simulink model "huizhenglijujisuan_zuixin"  (R2024b)
settings: Solver=FixedStepAuto  StartTime=0.0  StopTime=10  FixedStep=1e-4  MaxStep=1e-2  RelTol=1e-3
model workspace (MAT data in the model file):
  angle = Simulink.Parameter
  angle.Value = [-0.500377774 -0.503118992 -0.475854188 -0.406988144 -0.304092586 -0.178856105 -0.040153947 0.103196472 0.244897678 0.381538063 0.512861133 0.642340958 ... (2682 elements, 2682x1)]
  angle.Complexity = 'real'
  angle.Dimensions = [2682 1]
  angle.DataType = 'auto'
libraries: simulink x4, spsPermanentMagnetSynchronousMachineLib x2, slpidlib x2, powerlib_extras x2, Solver_SF x1, spsDCVoltageSourceLib x1, spsUniversalBridgeLib x1, spspowerguiLib x1
(part 1 of 2)
settings Model: Creator=L大锤  LastModifiedBy=L大锤
settings DataIOCC: ExternalInput=[t, a]
settings ModelReferenceCC: EnableRefExpFcnMdlSchedulingChecks=on
settings RTWCC: GPUComputeCapability=3.5

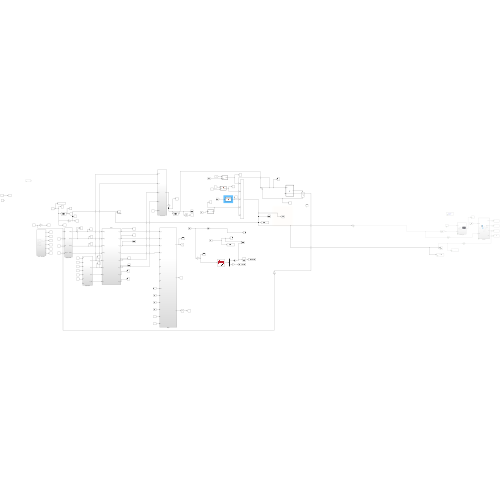
[thumbnail: Simulink's stored preview of the top-level diagram]
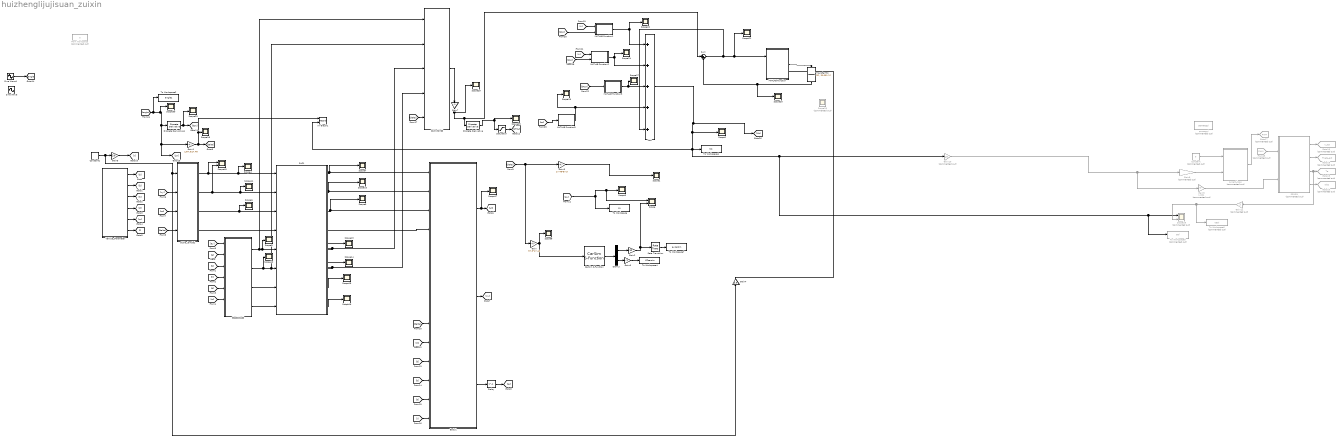
== system huizhenglijujisuan_zuixin ==
  Add : Sum  Inputs=+++++
  Body1 : Subsystem
  CarSim S-Function : Solver_SF/CarSim S-Function  Priority=1  SIMFILE=simfile.sim  Run_RTs=off  vs_state_ind=Run  StopMode_ind=Vehicle Model
  Constant : Constant  Commented=on  Value=0
  Constant1 : Constant  Value=80/3.6
  Delay : Delay  DelayLength=1
  Demux : Demux  Outputs=2
  Discrete Derivative : simulink/Quick Insert/Discrete/Discrete Derivative  gainval=1.0  ICPrevScaledInput=0.0  OutMin=[]  OutMax=[10]  OutDataType=fixdt(1, 16)  OutScaling=2^-10  DoSatur=on
  Discrete Derivative1 : simulink/Quick Insert/Discrete/Discrete Derivative  gainval=1.0  ICPrevScaledInput=0.0  OutMin=[]  OutMax=[]  OutDataType=fixdt(1, 16)  OutScaling=2^-10  DoSatur=off
  From Workspace : FromWorkspace  Commented=on  VariableName=a  OutDataTypeStr=double  SampleTime=0.001  Interpolate=off  OutputAfterFinalValue=Setting to zero
  From25 : From  Commented=on  GotoTag=PWM  TagVisibility=global
  Gain : Gain  Gain=57.3*17.48
  Gain1 : Gain  Gain=1/57.3/17.48
  Gain10 : Gain  Commented=on  Gain=1/3
  Gain11 : Gain  Commented=on  Gain=3
  Gain2 : Gain  Gain=10
  Gain3 : Gain  Gain=17.48*57.3
  Gain4 : Gain  Gain=3.6
  Gain5 : Gain  Gain=3.6
  Gain6 : Gain  Gain=-1
  Gain7 : Gain  Gain=-1
  Gain8 : Gain  Commented=on  Gain=1/0.11247
  Gain9 : Gain  Commented=on  Gain=1.001
  Goto15 : Goto  Commented=on  GotoTag=n_act  TagVisibility=global
  Goto16 : Goto  Commented=on  GotoTag=Iabc  TagVisibility=global
  Goto17 : Goto  Commented=on  GotoTag=PWM  TagVisibility=global
  Goto18 : Goto  Commented=on  GotoTag=Theta_act  TagVisibility=global
  Goto19 : Goto  Commented=on  GotoTag=Te  TagVisibility=global
  MATLAB Function : MATLAB Function  TreatAsAtomicUnit=on
  MATLAB Function1 : MATLAB Function  TreatAsAtomicUnit=on
  MATLAB Function2 : MATLAB Function  TreatAsAtomicUnit=on
  MATLAB Function3 : MATLAB Function  TreatAsAtomicUnit=on
  MATLAB Function5 : MATLAB Function  TreatAsAtomicUnit=on
  PAC1 : Subsystem
  Rate Transition : RateTransition
  SPMSM : Subsystem  Commented=on
  Saturation : Saturate  UpperLimit=10  LowerLimit=-10
  Scope : Scope  NumInputPorts=2
  Scope{1..25,27,29..30} (28 alike) : Scope
  Scope26 : Scope  Commented=on
  Scope28 : Scope  Commented=on  NumInputPorts=2
  Scope48 : Scope  NumInputPorts=2
  Sine Wave : Sin  Amplitude=400  Frequency=2*pi/10  SampleTime=0
  Sine Wave1 : Sin  Amplitude=20  Frequency=2*pi/5  SampleTime=0
  Sum : Sum  Inputs=|+-
  To Workspace : ToWorkspace  VariableName=ay  SampleTime=-1
  To Workspace1 : ToWorkspace  VariableName=MZ  SampleTime=-1
  To Workspace2 : ToWorkspace  VariableName=angle1  SampleTime=-1
  To Workspace4 : ToWorkspace  VariableName=MZcarsim  SampleTime=-1
  To Workspace5 : ToWorkspace  Commented=on  VariableName=tref  SampleTime=-1
  To Workspace6 : ToWorkspace  Commented=on  VariableName=treal  SampleTime=-1
  To Workspace7 : ToWorkspace  VariableName=aycarsim  SampleTime=-1
  Transfer Fcn : TransferFcn  Denominator=[0.001 1]
  Vehicle_Parameter : Subsystem
  XY Graph1 : Record  FileSettingsInternal="{\"entries\":[{\"content\":{\"excelSettings\":{\"content\":{},\"type\":\"Streamout.ExcelSettings\"}},\"type\":\"Streamout.FileSettingStorage\",\"uuid\":\"\"}],\"packageUris\":[\"http:\\/\\/schema.mathworks.com\\/mf0\\/streamout_blocks\\/R2020a\"],\"version\":\"1.0\"}"  Layout=[1 1]  SignalsInternal="{\"entries\":[{\"content\":{\"signals\":[{\"content\":{\"blockPath\":[],\"dimensions\":[1],\"domain\":\"\",\"lineColor\":\"#edb120\",\"lineWidth\":2,\"port\":1,\"sid\":[\"\"],\"signalID\":1,\"signalName\":\"Gain1\"},\"type\":\"RecordBlkView.Signal\",\"uuid\":\"\"},{\"content\":{\"blockPath\":[],\"dimensions\":[1],\"domain\":\"\",\"lineColor\":\"#7e2f8e\",\"lineWidth\":2,\"port\":2,\"sid\":[\"\"],\"signalID\":2,\"signalName\":\"Add\"},\"type\":\"RecordBlkView.Signal\",\"uuid\":\"\"}]},\"type\":\"RecordBlkView.InputSignals\",\"uuid\":\"\"}],\"packageUris\":[\"http:\\/\\/schema.mathworks.com\\/mf0\\/streamout_blocks\\/R2020a\"],\"version\":\"1.0\"}"  VisualizationBindings="{\"xyplotplugin\":{\"info\":[{\"series\":[],\"subplotID\":1}]}}"  CompatibilityTag=XY
  alpha_lamda1 : Subsystem
  current_loop : Subsystem  Commented=on
  powergui : spspowerguiLib/powergui  Priority=1  Commented=on  SimulationMode=Discrete  SampleTime=1/2000/500  frequency=60  Iterations=50  frequencyindice=0  Pbase=100e6  ErrMax=1e-4  UnitsV=kV  UnitsW=MW  buscounter=0  FunctionMessages=off  echomessages=off  EnableUseOfTLC=off  CurrentSourceSwitches=off  DisableSnubberDevices=off  DisableRonSwitches=off  DisableVfSwitches=off  DisplayEquations=off  AutomaticDiscreteSolvers=off  SolverType=Tustin/Backward Euler (TBE)  Interpol=off  ExternalGateDelay=off  methode=off  Ts=100  x0status=blocks  SPID=on  SwTol=0  HookPort=off  NonlinearTolerance=1e-4  nMaxIteration=100  ContinueOnMaxIteration=off  RestoreLinks=warning  ResistiveCurrentMeasurement=off  Frange=[0:2:500]  Ylog=off  Xlog=on  ShowGrid=off  save=off  variable=ZData  structure=ia  ZoomFFT=off  StartTime=.775  cycles=1  DisplayStyle=1  fundamental=400  FreqAxis=off  MaxFrequency=40000  frequencyindicesteady=1  RmsSteady=1  display=off
  回正力矩计算 : Subsystem
  垂直载荷估算 : Subsystem
  wires:
  alpha_lamda1/1(alpha_fl) -> Scope48/1, Scope4/1, PAC1/1(alpha_fl)
  alpha_lamda1/2(alpha_fr) -> Scope48/2, Scope11/1, PAC1/2(alpha_fr)
  alpha_lamda1/4(alpha_rr) -> PAC1/4(alpha_rr)
  垂直载荷估算/3(Fz_L2) -> PAC1/7(Fz_rl)
  垂直载荷估算/4(Fz_R2) -> PAC1/8(Fz_rr)
  垂直载荷估算/2(Fz_fr) -> 回正力矩计算/2(Fz_fr), PAC1/6(Fz_fr), Scope12/1
  垂直载荷估算/1(Fz_fl) -> 回正力矩计算/1(Fz_fl), PAC1/5(Fz_fl), Scope5/1
  PAC1/1(Fy_fl) -> Scope7/1, Body1/1(Fy_fl)
  PAC1/2(Fy_fr) -> Scope10/1, Body1/2(Fy_fr)
  PAC1/3(Fy_rl) -> Scope9/1, Body1/3(Fy_rl)
  PAC1/4(Fy_rr) -> Body1/4(Fy_rr)
  Gain/1 -> CarSim S-Function/1, Scope8/1
  PAC1/5(Mz_fl) -> Scope13/1, 回正力矩计算/3(M_fl)
  PAC1/6(Mz_fr) -> Scope14/1, 回正力矩计算/4(M_fr)
  Gain3/1 -> Scope1/1
  Body1/3(ay) -> Delay/1
  alpha_lamda1/3(alpha_rl) -> Scope6/1, PAC1/3(alpha_rl)
  PAC1/7(Mz_rl) -> Scope15/1
  PAC1/8(Mz_rr) -> Scope16/1
  Vehicle_Parameter/1(a) -> [a]
  Vehicle_Parameter/2(b) -> [b]
  Vehicle_Parameter/3(h) -> [h]
  Vehicle_Parameter/4(d) -> [d]
  Vehicle_Parameter/5(m) -> [m]
  Vehicle_Parameter/6(l) -> [I]
  [a] -> 垂直载荷估算/2(a)
  [b] -> 垂直载荷估算/3(b)
  [h] -> 垂直载荷估算/4(h)
  [d] -> 垂直载荷估算/5(d)
  [m] -> 垂直载荷估算/6(m)
  [ay] -> 垂直载荷估算/1(Ay)
  [vy] -> alpha_lamda1/2(vy)
  [wz] -> alpha_lamda1/3(wz)
  [delta] -> alpha_lamda1/4(delta_fl)
  Delay/1 -> [ay]
  Body1/2(vy) -> [vy]
  Body1/1(wz) -> Scope17/1, [wz]
  [delta] -> Gain3/1, Gain/1
  [delta] -> Body1/9(delta)
  [ay] -> Scope/1, Scope3/1, To Workspace/1
  [m] -> Body1/10(m)
  [d] -> Body1/11(d)
  [b] -> Body1/12(b)
  [a] -> Body1/13(a)
  [I] -> Body1/14(Iz)
  [delta] -> 回正力矩计算/5(delta)
  Gain1/1 -> XY Graph1/1, Scope18/1, [delta]
  Constant1/1 -> Gain4/1, alpha_lamda1/1(vx), Gain5/1
  Gain4/1 -> MATLAB Function/2(v)
  MATLAB Function/1(Tz) -> Transfer Fcn/1
  Transfer Fcn/1 -> Scope20/1, Sum/2
  Gain5/1 -> [v]
  Discrete Derivative1/1 -> [dsw], Scope23/1
  回正力矩计算/1(Mz) -> Gain7/1
  [sw] -> MATLAB Function5/1(sw)
  Demux/1 -> Gain2/1
  Demux/2 -> Gain6/1
  Gain7/1 -> Scope29/1, Discrete Derivative/1, Sum/1
  Gain6/1 -> To Workspace4/1
  [angle] -> To Workspace2/1, Scope30/1, Discrete Derivative1/1, [sw], Gain1/1
  MATLAB Function5/1(Tlim) -> Scope19/1, Add/4
  CarSim S-Function/1 -> Demux/1
  MATLAB Function3/1(Tguanxing) -> Scope27/1, Add/3
  [v] -> MATLAB Function2/1(v)
  [dsw] -> MATLAB Function2/2(dsw)
  [v] -> MATLAB Function1/1(v)
  MATLAB Function2/1(Tzuni) -> Scope24/1, Add/2
  [dsw] -> MATLAB Function1/2(dsw)
  MATLAB Function1/1(Tfric) -> Add/1, Scope22/1
  [dTsw] -> MATLAB Function3/1(dtsw)
  Sum/1 -> Scope21/1, MATLAB Function/1(Tsw), Add/5
  Discrete Derivative/1 -> Saturation/1, Scope25/1
  Saturation/1 -> [dTsw]
  From25/1 -> SPMSM/1(pwm)
  SPMSM/2(theta_act) -> Goto18/1
  current_loop/1(pwm) -> Goto17/1
  Gain9/1 -> SPMSM/2(load)
  Gain8/1 -> current_loop/2(iq*)
  SPMSM/4(Iabc) -> Goto16/1
  SPMSM/1(n_act) -> Goto15/1
  Constant/1 -> current_loop/1(id*)
  Add/1 -> [Mz], To Workspace5/1, Scope28/1, Gain10/1, XY Graph1/2, To Workspace1/1, Scope2/1
  SPMSM/3(Te) -> Gain11/1, Goto19/1
  Gain10/1 -> Gain9/1, Gain8/1
  Gain11/1 -> To Workspace6/1, Scope28/2
  Gain2/1 -> Rate Transition/1, Scope/2
  Sine Wave1/1 -> [angle]
  Rate Transition/1 -> To Workspace7/1

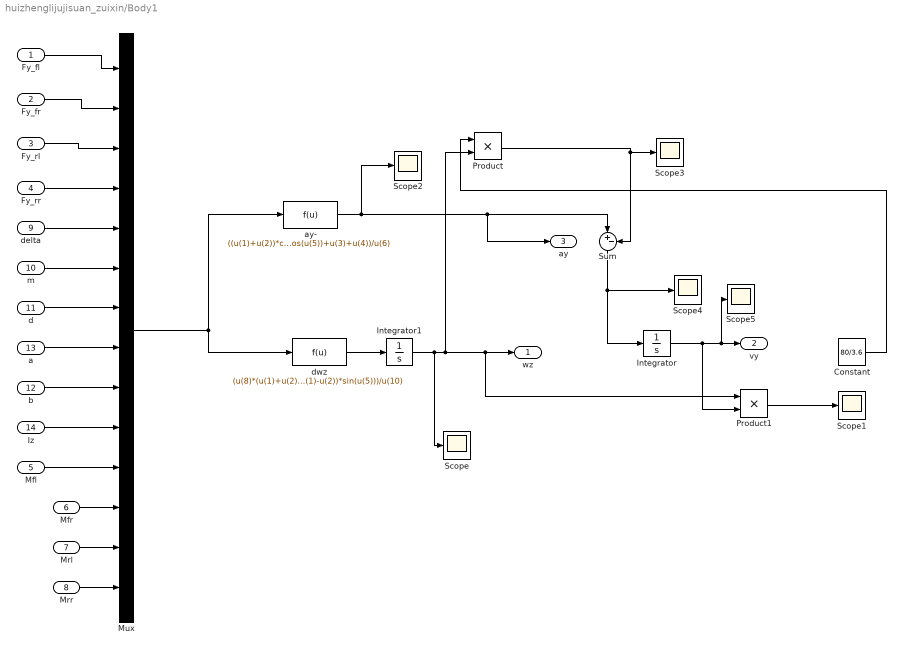
== system huizhenglijujisuan_zuixin/Body1 ==
  Fy_fl : Inport
  Fy_fr : Inport  Port=2
  Fy_rl : Inport  Port=3
  Fy_rr : Inport  Port=4
  Mfl : Inport  Port=5
  Mfr : Inport  Port=6
  Mrl : Inport  Port=7
  Mrr : Inport  Port=8
  delta : Inport  Port=9
  m : Inport  Port=10
  d : Inport  Port=11
  b : Inport  Port=12
  a : Inport  Port=13
  Iz : Inport  Port=14
  Constant : Constant  Value=80/3.6
  Integrator : Integrator
  Integrator1 : Integrator
  Mux : Mux  Inputs=14
  Product : Product
  Product1 : Product
  Scope{,1..5} (6 alike) : Scope
  Sum : Sum  Inputs=|+-
  ay- : Fcn  Expr=((u(1)+u(2))*cos(u(5))+u(3)+u(4))/u(6)
  dwz : Fcn  Expr=(u(8)*(u(1)+u(2))*cos(u(5))-u(9)*(u(3)+u(4))+u(7)/2*(u(1)-u(2))*sin(u(5)))/u(10)
  wz : Outport
  vy : Outport  Port=2
  ay : Outport  Port=3
  wires:
  Mux/1 -> ay-/1, dwz/1
  ay-/1 -> Scope2/1, ay/1, Sum/1
  dwz/1 -> Integrator1/1
  Integrator1/1 -> Scope/1, Product/2, Product1/1, wz/1
  Fy_fl/1 -> Mux/1
  Fy_fr/1 -> Mux/2
  Fy_rl/1 -> Mux/3
  Fy_rr/1 -> Mux/4
  delta/1 -> Mux/5
  m/1 -> Mux/6
  Constant/1 -> Product/1
  Product/1 -> Scope3/1, Sum/2
  Sum/1 -> Scope4/1, Integrator/1
  Integrator/1 -> Product1/2, Scope5/1, vy/1
  Product1/1 -> Scope1/1
  d/1 -> Mux/7
  a/1 -> Mux/8
  b/1 -> Mux/9
  Iz/1 -> Mux/10
  Mfl/1 -> Mux/11
  Mfr/1 -> Mux/12
  Mrl/1 -> Mux/13
  Mrr/1 -> Mux/14

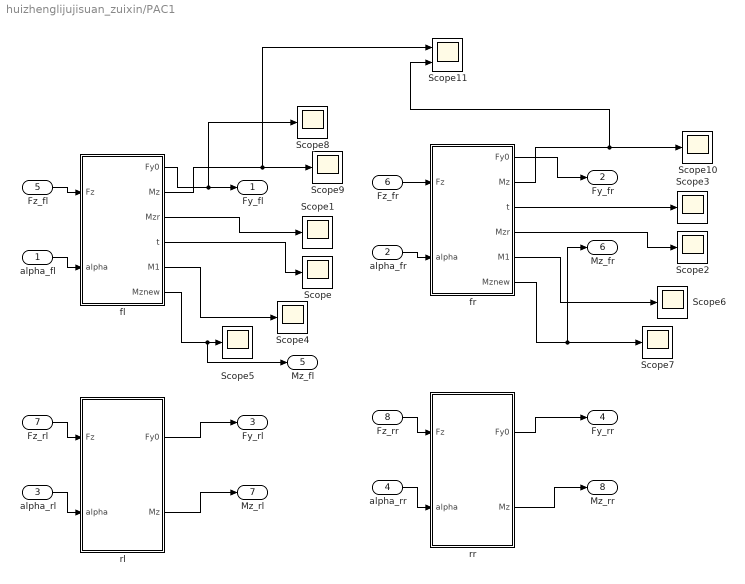
== system huizhenglijujisuan_zuixin/PAC1 ==
  alpha_fl : Inport
  alpha_fr : Inport  Port=2
  alpha_rl : Inport  Port=3
  alpha_rr : Inport  Port=4
  Fz_fl : Inport  Port=5
  Fz_fr : Inport  Port=6
  Fz_rl : Inport  Port=7
  Fz_rr : Inport  Port=8
  Scope{,1..10} (11 alike) : Scope
  Scope11 : Scope  NumInputPorts=2
  fl : MATLAB Function  TreatAsAtomicUnit=on
  fr : MATLAB Function  TreatAsAtomicUnit=on
  rl : MATLAB Function  TreatAsAtomicUnit=on
  rr : MATLAB Function  TreatAsAtomicUnit=on
  Fy_fl : Outport
  Fy_fr : Outport  Port=2
  Fy_rl : Outport  Port=3
  Fy_rr : Outport  Port=4
  Mz_fl : Outport  Port=5
  Mz_fr : Outport  Port=6
  Mz_rl : Outport  Port=7
  Mz_rr : Outport  Port=8
  wires:
  fl/2(Mz) -> Scope11/1, Scope9/1
  Fz_fl/1 -> fl/1(Fz)
  alpha_fl/1 -> fl/2(alpha)
  fl/1(Fy0) -> Scope8/1, Fy_fl/1
  Fz_fr/1 -> fr/1(Fz)
  alpha_fr/1 -> fr/2(alpha)
  fr/1(Fy0) -> Fy_fr/1
  Fz_rl/1 -> rl/1(Fz)
  alpha_rl/1 -> rl/2(alpha)
  rl/1(Fy0) -> Fy_rl/1
  Fz_rr/1 -> rr/1(Fz)
  alpha_rr/1 -> rr/2(alpha)
  rr/2(Mz) -> Mz_rr/1
  rr/1(Fy0) -> Fy_rr/1
  fl/4(t) -> Scope/1
  fl/3(Mzr) -> Scope1/1
  fr/4(Mzr) -> Scope2/1
  fr/3(t) -> Scope3/1
  fl/5(M1) -> Scope4/1
  fl/6(Mznew) -> Mz_fl/1, Scope5/1
  fr/5(M1) -> Scope6/1
  fr/6(Mznew) -> Mz_fr/1, Scope7/1
  fr/2(Mz) -> Scope11/2, Scope10/1
  rl/2(Mz) -> Mz_rl/1

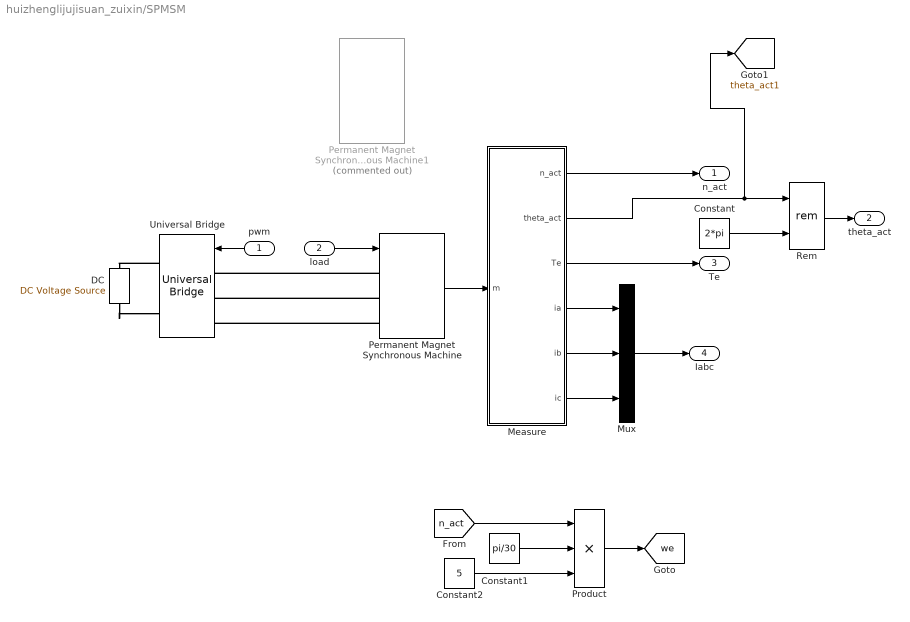
== system huizhenglijujisuan_zuixin/SPMSM ==
  pwm : Inport
  load : Inport  Port=2
  Constant : Constant  Value=2*pi
  Constant1 : Constant  Value=pi/30
  Constant2 : Constant  Value=5
  "DC " : spsDCVoltageSourceLib/DC Voltage Source  Amplitude=200  Measurements=None
  Measure : Subsystem
  Mux : Mux  Inputs=3
  Permanent Magnet Synchronous Machine : spsPermanentMagnetSynchronousMachineLib/Permanent Magnet Synchronous Machine  NbPhases=3  FluxDistribution=Sinusoidal  RotorType=Round  MechanicalLoad=Torque Tm  PresetModel=No  ShowDetailedParameters=on  MeasurementBus=off  Resistance=0.12  Inductance=8.5e-3  dqInductances=[4e-3, 4e-3]  La=0.97e-3  MachineConstant=Voltage Constant (V_peak L-L / krpm)  Flux=0.014996  VoltageCst=13.6  TorqueCst=0.11247  Flat=120  Mechanical=[0.00107 0 5 0]  PolePairs=4  InitialConditions=[0,0, 0,0]  InitialConditions5ph=[0 0 0 0 0 0]  RefAngle=Aligned with phase A axis (original Park)  IterativeDiscreteModel=Trapezoidal non iterative  TsBlock=-1  TsPowergui=0
  Permanent Magnet Synchronous Machine1 : spsPermanentMagnetSynchronousMachineLib/Permanent Magnet Synchronous Machine  Commented=on  NbPhases=3  FluxDistribution=Sinusoidal  RotorType=Salient-pole  MechanicalLoad=Torque Tm  PresetModel=No  ShowDetailedParameters=on  MeasurementBus=off  Resistance=2.875  Inductance=8.5e-3  dqInductances=[4e-3, 4e-3]  La=0.000835  MachineConstant=Flux linkage established by magnets (V.s)  Flux=0.175  VoltageCst=126.966  TorqueCst=1.05  Flat=120  Mechanical=[0.003 0 4 0]  PolePairs=4  InitialConditions=[0,0, 0,0]  InitialConditions5ph=[0 0 0 0 0 0]  RefAngle=Aligned with phase A axis (original Park)  IterativeDiscreteModel=Trapezoidal non iterative  TsBlock=-1  TsPowergui=0
  Product : Product  Inputs=3
  Rem : Math  Operator=rem
  Universal Bridge : spsUniversalBridgeLib/Universal Bridge  Arms=3  SnubberResistance=1e5  SnubberCapacitance=inf  Device=IGBT / Diodes  Ron=1e-3  Lon=0  ForwardVoltages="[  0  0  ]"  ForwardVoltage=0  GTOparameters=[ 10e-6 , 20e-6 ]  IGBTparameters=[ 1e-6 , 2e-6 ]  Measurements=None  Measurements_2=None  converterType=Rectifier
  n_act : Outport
  theta_act : Outport  Port=2
  Te : Outport  Port=3
  Iabc : Outport  Port=4
  tag scope: theta_act1=global, we=global
  wires:
  pwm/1 -> Universal Bridge/1
  load/1 -> Permanent Magnet Synchronous Machine/1
  Permanent Magnet Synchronous Machine/1 -> Measure/1(m)
  Measure/1(n_act) -> n_act/1
  Measure/3(Te) -> Te/1
  Measure/4(ia) -> Mux/1
  Measure/5(ib) -> Mux/2
  Measure/6(ic) -> Mux/3
  Mux/1 -> Iabc/1
  Rem/1 -> theta_act/1
  Constant/1 -> Rem/2
  Measure/2(theta_act) -> [theta_act1], Rem/1
  [n_act] -> Product/1
  Constant1/1 -> Product/2
  Constant2/1 -> Product/3
  Product/1 -> [we]
  connections:
  "DC "/LConn1 -- Universal Bridge/RConn2
  Universal Bridge/RConn1 -- "DC "/RConn1
  Permanent Magnet Synchronous Machine/LConn3 -- Universal Bridge/LConn3
  Permanent Magnet Synchronous Machine/LConn1 -- Universal Bridge/LConn1
  Permanent Magnet Synchronous Machine/LConn2 -- Universal Bridge/LConn2

== system huizhenglijujisuan_zuixin/Vehicle_Parameter ==
  Constant : Constant  Value=2636
  Constant1 : Constant  Value=1.701
  Constant2 : Constant  Value=1.427
  Constant3 : Constant  Value=1.572
  Constant4 : Constant  Value=0.5848
  Constant8 : Constant  Value=4500
  a : Outport
  b : Outport  Port=2
  h : Outport  Port=3
  d : Outport  Port=4
  m : Outport  Port=5
  l : Outport  Port=6
  wires:
  Constant/1 -> m/1
  Constant3/1 -> a/1
  Constant2/1 -> b/1
  Constant4/1 -> h/1
  Constant1/1 -> d/1
  Constant8/1 -> l/1

== system huizhenglijujisuan_zuixin/alpha_lamda1 ==
  vx : Inport
  vy : Inport  Port=2
  wz : Inport  Port=3
  delta_fl : Inport  Port=4
  alpha : Subsystem
  alpha_fl : Outport
  alpha_fr : Outport  Port=2
  alpha_rl : Outport  Port=3
  alpha_rr : Outport  Port=4
  wires:
  alpha/1(alpha_fl) -> alpha_fl/1
  alpha/2(alpha_fr) -> alpha_fr/1
  alpha/3(alpha_rl) -> alpha_rl/1
  alpha/4(alpha_rr) -> alpha_rr/1
  vx/1 -> alpha/1(vx)
  vy/1 -> alpha/2(vy)
  wz/1 -> alpha/3(wz)
  delta_fl/1 -> alpha/4(delta_fl)

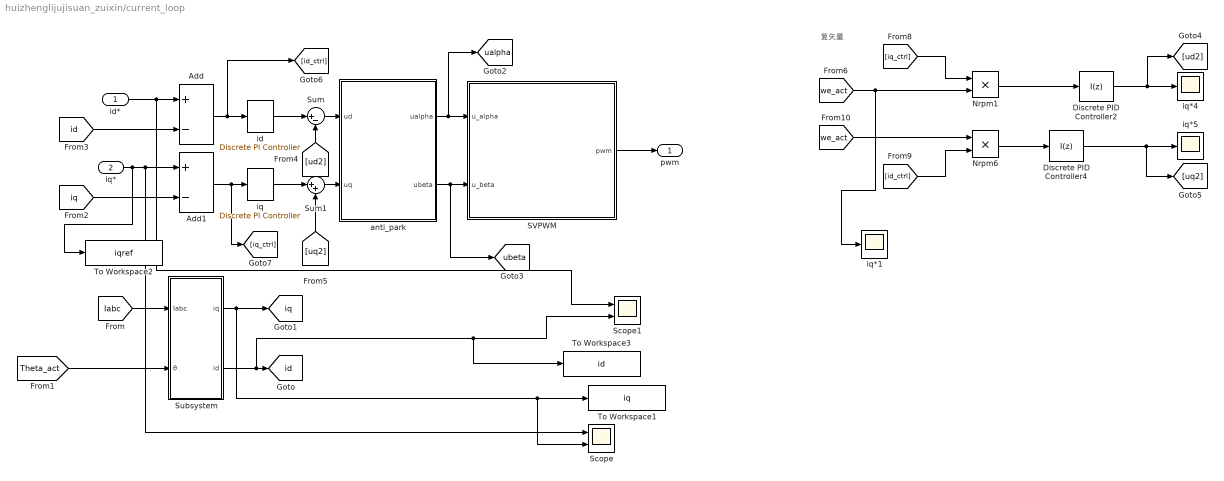
== system huizhenglijujisuan_zuixin/current_loop ==
  note: 复矢量
  id* : Inport
  iq* : Inport  Port=2
  Add : Sum  Inputs=+-
  Add1 : Sum  Inputs=+-
  Discrete PID Controller2 : slpidlib/PID Controller  Controller=I  Form=Parallel  TimeDomain=Discrete-time  UseExternalTs=off  SampleTime=1e-4  IntegratorMethod=Forward Euler  FilterMethod=Forward Euler  ControllerParametersSource=internal  P=0  I=0.32/10000  UseKiTs=off  D=0  UseExternalDerivativeSource=off  N=100  UseFilter=on  TunerSelectOption=Transfer Function Based (PID Tuner App)  InitialConditionSource=internal  InitialConditionForIntegrator=0  InitialConditionForFilter=0  DifferentiatorICPrevScaledInput=0  ExternalReset=none  TrackingMode=off  Kt=1  LimitOutput=on  SatLimitsSource=internal  UpperSaturationLimit=600  LowerSaturationLimit=-600  LinearizeAsGain=off  AntiWindupMode=none  Kb=1  LimitIntegrator=off  UpperIntegratorSaturationLimit=inf  LowerIntegratorSaturationLimit=-inf  POutMin=[]  POutMax=[]  IOutMin=[]  IOutMax=[]  DOutMin=[]  DOutMax=[]  NOutMin=[]  NOutMax=[]  SumOutMin=[]  SumOutMax=[]  SaturationOutMin=[]  SaturationOutMax=[]  PParamMin=[]  PParamMax=[]  IParamMin=[]  IParamMax=[]  DParamMin=[]  DParamMax=[]  NParamMin=[]  NParamMax=[]  KbParamMin=[]  KbParamMax=[]  KtParamMin=[]  KtParamMax=[]  KbOutMin=[]  KbOutMax=[]  KtOutMin=[]  KtOutMax=[]  IntegratorOutMin=[]  IntegratorOutMax=[]  FilterOutMin=[]  FilterOutMax=[]  SumI1OutMin=[]  SumI1OutMax=[]  SumI2OutMin=[]  SumI2OutMax=[]  SumI3OutMin=[]  SumI3OutMax=[]  SumI4OutMin=[]  SumI4OutMax=[]  SumDOutMin=[]  SumDOutMax=[]  DifferentiatorOutMin=[]  DifferentiatorOutMax=[]  FilterDiffOutCoefMin=[]  FilterDiffOutCoefMax=[]  ReciprocalOutMin=[]  ReciprocalOutMax=[]  SumDenOutMin=[]  SumDenOutMax=[]  SumNumOutMin=[]  SumNumOutMax=[]  DivideOutMin=[]  DivideOutMax=[]  UdiffTsProdOutMin=[]  UdiffTsProdOutMax=[]  NTsProdOutMin=[]  NTsProdOutMax=[]  UintegralTsProdOutMin=[]  UintegralTsProdOutMax=[]  UngainTsProdOutMin=[]  UngainTsProdOutMax=[]  ClampingZeroOutDataTypeStr=Inherit: Inherit via back propagation  ClampingZeroOutMin=[]  ClampingZeroOutMax=[]  FilterDenConstantOutDataTypeStr=Inherit: Inherit via back propagation  FilterDenConstantOutMin=[]  FilterDenConstantOutMax=[]  PCopyOutDataTypeStr=Inherit: Inherit via back propagation  PCopyOutMin=[]  PCopyOutMax=[]  NCopyOutDataTypeStr=Inherit: Inherit via back propagation  NCopyOutMin=[]  NCopyOutMax=[]  IntegratorContinuousStateAttributes=''  IntegratorStateMustResolveToSignalObject=off  IntegratorRTWStateStorageClass=Auto  FilterContinuousStateAttributes=''  FilterStateMustResolveToSignalObject=off  FilterRTWStateStorageClass=Auto  ParallelPVariant=Disabled  IdealPVariant=Disabled  IVariant=InternalParameters  DVariant=Disabled  IntegratorVariant=Discrete  SatVariant=Enabled  AWVariant=Passthrough  PCopyVariant=Disabled  TRVariant=Disabled  FdbkBlocksVariant=Forward  IdealPFdbkVariant=Disabled  SatFdbkVariant=Disabled  DerivativeFilterVariant=Disabled  NVariant=Disabled  NCopyVariant=Disabled_SignalSpec  FilterICVariant=Disabled  IntegratorICVariant=InternalICs  ExternalResetVariant=Disabled  TRSumVariant=Passthrough  SumFdbkVariant=Disabled  SumVariant=Passthrough_I  TsampFilterVariant=InternalTs  TsampNgainVariant=Passthrough  TsampIntegralVariant=Disabled_SignalSpec  ExternalSaturationOutDataTypeStr=Inherit: Same as second input  DerivativeSourceVariant=Disabled  PreIntVariant=InternalPreInt
  Discrete PID Controller4 : slpidlib/PID Controller  Controller=I  Form=Parallel  TimeDomain=Discrete-time  UseExternalTs=off  SampleTime=1e-4  IntegratorMethod=Forward Euler  FilterMethod=Forward Euler  ControllerParametersSource=internal  P=0  I=0.32/10000  UseKiTs=off  D=0  UseExternalDerivativeSource=off  N=100  UseFilter=on  TunerSelectOption=Transfer Function Based (PID Tuner App)  InitialConditionSource=internal  InitialConditionForIntegrator=0  InitialConditionForFilter=0  DifferentiatorICPrevScaledInput=0  ExternalReset=none  TrackingMode=off  Kt=1  LimitOutput=on  SatLimitsSource=internal  UpperSaturationLimit=600  LowerSaturationLimit=-600  LinearizeAsGain=off  AntiWindupMode=none  Kb=1  LimitIntegrator=off  UpperIntegratorSaturationLimit=inf  LowerIntegratorSaturationLimit=-inf  POutMin=[]  POutMax=[]  IOutMin=[]  IOutMax=[]  DOutMin=[]  DOutMax=[]  NOutMin=[]  NOutMax=[]  SumOutMin=[]  SumOutMax=[]  SaturationOutMin=[]  SaturationOutMax=[]  PParamMin=[]  PParamMax=[]  IParamMin=[]  IParamMax=[]  DParamMin=[]  DParamMax=[]  NParamMin=[]  NParamMax=[]  KbParamMin=[]  KbParamMax=[]  KtParamMin=[]  KtParamMax=[]  KbOutMin=[]  KbOutMax=[]  KtOutMin=[]  KtOutMax=[]  IntegratorOutMin=[]  IntegratorOutMax=[]  FilterOutMin=[]  FilterOutMax=[]  SumI1OutMin=[]  SumI1OutMax=[]  SumI2OutMin=[]  SumI2OutMax=[]  SumI3OutMin=[]  SumI3OutMax=[]  SumI4OutMin=[]  SumI4OutMax=[]  SumDOutMin=[]  SumDOutMax=[]  DifferentiatorOutMin=[]  DifferentiatorOutMax=[]  FilterDiffOutCoefMin=[]  FilterDiffOutCoefMax=[]  ReciprocalOutMin=[]  ReciprocalOutMax=[]  SumDenOutMin=[]  SumDenOutMax=[]  SumNumOutMin=[]  SumNumOutMax=[]  DivideOutMin=[]  DivideOutMax=[]  UdiffTsProdOutMin=[]  UdiffTsProdOutMax=[]  NTsProdOutMin=[]  NTsProdOutMax=[]  UintegralTsProdOutMin=[]  UintegralTsProdOutMax=[]  UngainTsProdOutMin=[]  UngainTsProdOutMax=[]  ClampingZeroOutDataTypeStr=Inherit: Inherit via back propagation  ClampingZeroOutMin=[]  ClampingZeroOutMax=[]  FilterDenConstantOutDataTypeStr=Inherit: Inherit via back propagation  FilterDenConstantOutMin=[]  FilterDenConstantOutMax=[]  PCopyOutDataTypeStr=Inherit: Inherit via back propagation  PCopyOutMin=[]  PCopyOutMax=[]  NCopyOutDataTypeStr=Inherit: Inherit via back propagation  NCopyOutMin=[]  NCopyOutMax=[]  IntegratorContinuousStateAttributes=''  IntegratorStateMustResolveToSignalObject=off  IntegratorRTWStateStorageClass=Auto  FilterContinuousStateAttributes=''  FilterStateMustResolveToSignalObject=off  FilterRTWStateStorageClass=Auto  ParallelPVariant=Disabled  IdealPVariant=Disabled  IVariant=InternalParameters  DVariant=Disabled  IntegratorVariant=Discrete  SatVariant=Enabled  AWVariant=Passthrough  PCopyVariant=Disabled  TRVariant=Disabled  FdbkBlocksVariant=Forward  IdealPFdbkVariant=Disabled  SatFdbkVariant=Disabled  DerivativeFilterVariant=Disabled  NVariant=Disabled  NCopyVariant=Disabled_SignalSpec  FilterICVariant=Disabled  IntegratorICVariant=InternalICs  ExternalResetVariant=Disabled  TRSumVariant=Passthrough  SumFdbkVariant=Disabled  SumVariant=Passthrough_I  TsampFilterVariant=InternalTs  TsampNgainVariant=Passthrough  TsampIntegralVariant=Disabled_SignalSpec  ExternalSaturationOutDataTypeStr=Inherit: Same as second input  DerivativeSourceVariant=Disabled  PreIntVariant=InternalPreInt
  Nrpm1 : Product
  Nrpm6 : Product
  SVPWM : Subsystem
  Scope : Scope  NumInputPorts=2
  Scope1 : Scope  NumInputPorts=2
  Subsystem : Subsystem
  Sum : Sum  Inputs=|+-
  Sum1 : Sum  Inputs=|++
  To Workspace1 : ToWorkspace  VariableName=iq  SampleTime=-1
  To Workspace2 : ToWorkspace  VariableName=iqref  SampleTime=-1
  To Workspace3 : ToWorkspace  VariableName=id  SampleTime=-1
  anti_park : Subsystem
  id : powerlib_extras/Discrete  Control Blocks/Discrete PI Controller  Kp=0.32*2  Ki=0.004*2  Par_Limits=[200/1.732 -200/1.732]  Init=0  Ts=1e-4
  iq : powerlib_extras/Discrete  Control Blocks/Discrete PI Controller  Kp=0.32*2  Ki=0.004*2  Par_Limits=[200/1.732 -200/1.732]  Init=0  Ts=1e-4
  iq*1 : Scope
  iq*4 : Scope
  iq*5 : Scope
  pwm : Outport
  tag scope: id=global, iq=global, ualpha=global, ubeta=global
  wires:
  id*/1 -> Scope1/1, Add/1
  Add/1 -> [id_ctrl], id/1
  iq*/1 -> To Workspace2/1, Scope/1, Add1/1
  Add1/1 -> [iq_ctrl], iq/1
  anti_park/1(ualpha) -> [ualpha], SVPWM/1(u_alpha)
  anti_park/2(ubeta) -> [ubeta], SVPWM/2(u_beta)
  SVPWM/1(pwm) -> pwm/1
  [Iabc] -> Subsystem/1(Iabc)
  [iq] -> Add1/2
  [id] -> Add/2
  [Theta_act] -> Subsystem/2(θ)
  [ud2] -> Sum/2
  [uq2] -> Sum1/2
  id/1 -> Sum/1
  Sum/1 -> anti_park/1(ud)
  iq/1 -> Sum1/1
  Sum1/1 -> anti_park/2(uq)
  [id_ctrl] -> Nrpm6/2
  Nrpm1/1 -> Discrete PID Controller2/1
  Nrpm6/1 -> Discrete PID Controller4/1
  Discrete PID Controller2/1 -> [ud2], iq*4/1
  [we_act] -> iq*1/1, Nrpm1/2
  [we_act] -> Nrpm6/1
  Discrete PID Controller4/1 -> iq*5/1, [uq2]
  [iq_ctrl] -> Nrpm1/1
  Subsystem/2(id) -> To Workspace3/1, Scope1/2, [id]
  Subsystem/1(iq) -> To Workspace1/1, Scope/2, [iq]

== system huizhenglijujisuan_zuixin/回正力矩计算 ==
  Fz_fl : Inport
  Fz_fr : Inport  Port=2
  M_fl : Inport  Port=3
  M_fr : Inport  Port=4
  delta : Inport  Port=5
  Mhuizheng : Fcn  Expr=((u(1)+u(2))/2*0.0105*sin(2*13.2*pi/180)*sin(u(5)))/17.48
  Mhuizheng1 : Fcn  Expr=(u(3)+u(4))/17.48
  Mux : Mux  Inputs=5
  Scope : Scope
  Scope1 : Scope
  Sum : Sum  Inputs=|-+
  Mz : Outport
  wires:
  Fz_fl/1 -> Mux/1
  Fz_fr/1 -> Mux/2
  M_fl/1 -> Mux/3
  M_fr/1 -> Mux/4
  delta/1 -> Mux/5
  Mux/1 -> Mhuizheng1/1, Mhuizheng/1
  Mhuizheng1/1 -> Scope1/1, Sum/2
  Mhuizheng/1 -> Scope/1, Sum/1
  Sum/1 -> Mz/1

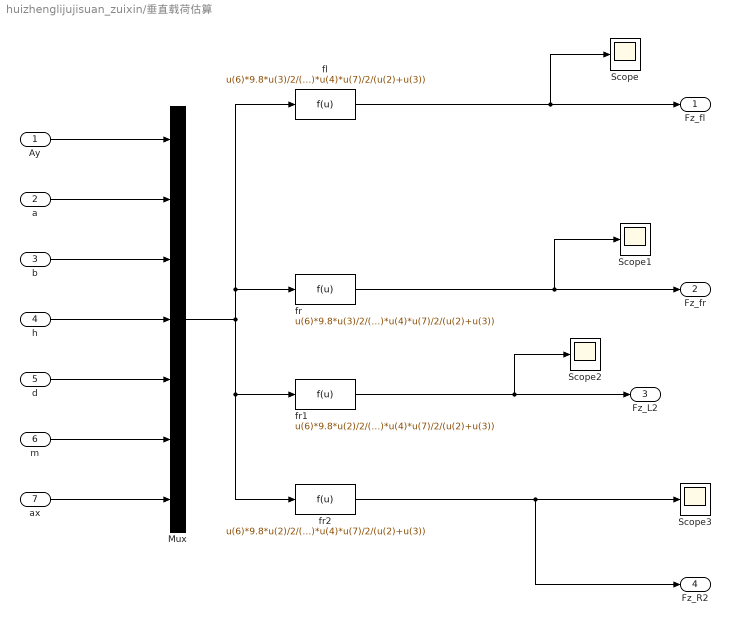
== system huizhenglijujisuan_zuixin/垂直载荷估算 ==
  Ay : Inport
  a : Inport  Port=2
  b : Inport  Port=3
  h : Inport  Port=4
  d : Inport  Port=5
  m : Inport  Port=6
  ax : Inport  Port=7
  Mux : Mux  Inputs=7
  Scope{,1..3} (4 alike) : Scope
  fl : Fcn  Expr=u(6)*9.8*u(3)/2/(u(2)+u(3))-u(6)*u(4)*u(3)*u(1)/u(5)/(u(2)+u(3))-u(6)*u(4)*u(7)/2/(u(2)+u(3))
  fr : Fcn  Expr=u(6)*9.8*u(3)/2/(u(2)+u(3))+u(6)*u(4)*u(3)*u(1)/u(5)/(u(2)+u(3))-u(6)*u(4)*u(7)/2/(u(2)+u(3))
  fr1 : Fcn  Expr=u(6)*9.8*u(2)/2/(u(2)+u(3))-u(6)*u(4)*u(2)*u(1)/u(5)/(u(2)+u(3))+u(6)*u(4)*u(7)/2/(u(2)+u(3))
  fr2 : Fcn  Expr=u(6)*9.8*u(2)/2/(u(2)+u(3))+u(6)*u(4)*u(2)*u(1)/u(5)/(u(2)+u(3))+u(6)*u(4)*u(7)/2/(u(2)+u(3))
  Fz_fl : Outport
  Fz_fr : Outport  Port=2
  Fz_L2 : Outport  Port=3
  Fz_R2 : Outport  Port=4
  wires:
  m/1 -> Mux/6
  h/1 -> Mux/4
  a/1 -> Mux/2
  Ay/1 -> Mux/1
  b/1 -> Mux/3
  d/1 -> Mux/5
  Mux/1 -> fr/1, fl/1, fr2/1, fr1/1
  fl/1 -> Scope/1, Fz_fl/1
  fr/1 -> Scope1/1, Fz_fr/1
  fr1/1 -> Scope2/1, Fz_L2/1
  fr2/1 -> Scope3/1, Fz_R2/1
  ax/1 -> Mux/7

== system huizhenglijujisuan_zuixin/SPMSM/Measure ==
  m : Inport
  Bus Selector : BusSelector  OutputSignals=Rotor speed wm (rad/s),Rotor angle thetam (rad),Electromagnetic torque Te (N*m),Stator current is_a (A),Stator current is_b (A),Stator current is_c (A)
  Gain : Gain  Gain=5
  Gain1 : Gain  Gain=30/pi
  P : Gain  Gain=5
  n_act : Outport  VectorParamsAs1DForOutWhenUnconnected=off
  theta_act : Outport  Port=2  VectorParamsAs1DForOutWhenUnconnected=off
  Te : Outport  Port=3  VectorParamsAs1DForOutWhenUnconnected=off
  ia : Outport  Port=4  VectorParamsAs1DForOutWhenUnconnected=off
  ib : Outport  Port=5  VectorParamsAs1DForOutWhenUnconnected=off
  ic : Outport  Port=6  VectorParamsAs1DForOutWhenUnconnected=off
  tag scope: we_act=global
  wires:
  m/1 -> Bus Selector/1
  Bus Selector/3 -> Te/1  "<Electromagnetic torque Te (N*m)>"
  Bus Selector/1 -> Gain/1, Gain1/1  "<Rotor speed wm (rad/s)>"
  Bus Selector/2 -> P/1  "<Rotor angle thetam (rad)>"
  Bus Selector/5 -> ib/1  "<Stator current is_b (A)>"
  Bus Selector/6 -> ic/1  "<Stator current is_c (A)>"
  P/1 -> theta_act/1
  Gain1/1 -> n_act/1
  Bus Selector/4 -> ia/1  "<Stator current is_a (A)>"
  Gain/1 -> [we_act]

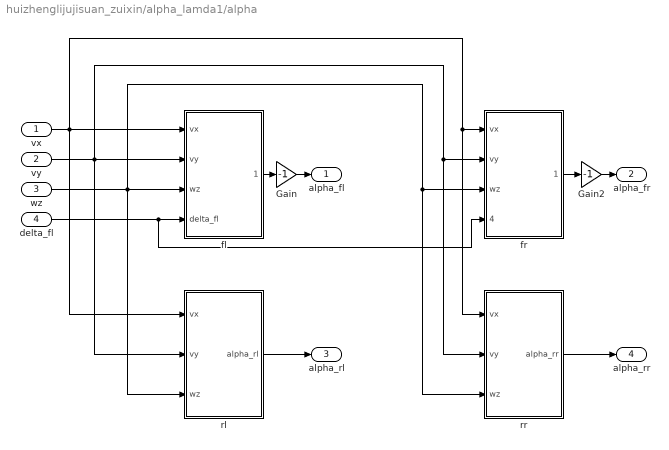
== system huizhenglijujisuan_zuixin/alpha_lamda1/alpha ==
  vx : Inport
  vy : Inport  Port=2
  wz : Inport  Port=3
  delta_fl : Inport  Port=4
  Gain : Gain  Gain=-1
  Gain2 : Gain  Gain=-1
  fl : Subsystem
  fr : Subsystem
  rl : Subsystem
  rr : Subsystem
  alpha_fl : Outport
  alpha_fr : Outport  Port=2
  alpha_rl : Outport  Port=3
  alpha_rr : Outport  Port=4
  wires:
  rr/1(alpha_rr) -> alpha_rr/1
  Gain2/1 -> alpha_fr/1
  fr/1(alpha_fr) -> Gain2/1
  rl/1(alpha_rl) -> alpha_rl/1
  Gain/1 -> alpha_fl/1
  fl/1(alpha_fl) -> Gain/1
  wz/1 -> fl/3(wz), rr/3(wz), fr/3(wz), rl/3(wz)
  vx/1 -> rr/1(vx), fr/1(vx), fl/1(vx), rl/1(vx)
  vy/1 -> rr/2(vy), fr/2(vy), fl/2(vy), rl/2(vy)
  delta_fl/1 -> fr/4(delta_fr), fl/4(delta_fl)

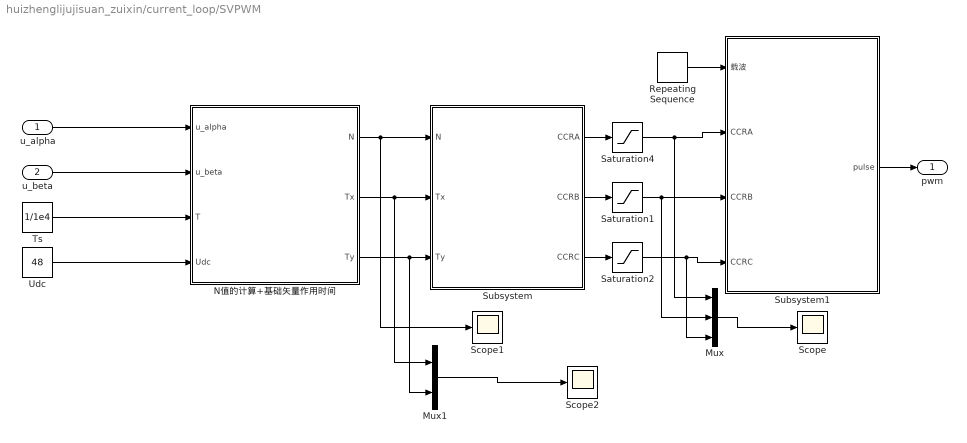
== system huizhenglijujisuan_zuixin/current_loop/SVPWM ==
  u_alpha : Inport
  u_beta : Inport  Port=2
  Mux : Mux  Inputs=3
  Mux1 : Mux  Inputs=2
  N值的计算+基础矢量作用时间 : Subsystem
  Repeating Sequence : simulink/Sources/Repeating Sequence  rep_seq_t=[0 1/1e4/2 1/1e4]  rep_seq_y=[0 1/1e4/2 0]
  Saturation1 : Saturate  UpperLimit=1/1e4/2  LowerLimit=0
  Saturation2 : Saturate  UpperLimit=1/1e4/2  LowerLimit=0
  Saturation4 : Saturate  UpperLimit=1/1e4/2  LowerLimit=0
  Scope : Scope
  Scope1 : Scope
  Scope2 : Scope
  Subsystem : Subsystem
  Subsystem1 : Subsystem
  Ts : Constant  Value=1/1e4
  Udc : Constant  Value=48
  pwm : Outport
  wires:
  Repeating Sequence/1 -> Subsystem1/1(载波)
  Subsystem1/1(pulse) -> pwm/1
  N值的计算+基础矢量作用时间/3(Ty) -> Mux1/2, Subsystem/3(Ty)
  N值的计算+基础矢量作用时间/2(Tx) -> Mux1/1, Subsystem/2(Tx)
  N值的计算+基础矢量作用时间/1(N) -> Scope1/1, Subsystem/1(N)
  Udc/1 -> N值的计算+基础矢量作用时间/4(Udc)
  Ts/1 -> N值的计算+基础矢量作用时间/3(T)
  u_beta/1 -> N值的计算+基础矢量作用时间/2(u_beta)
  u_alpha/1 -> N值的计算+基础矢量作用时间/1(u_alpha)
  Subsystem/2(CCRB) -> Saturation1/1
  Subsystem/3(CCRC) -> Saturation2/1
  Subsystem/1(CCRA) -> Saturation4/1
  Mux/1 -> Scope/1
  Saturation4/1 -> Mux/1, Subsystem1/2(CCRA)
  Saturation1/1 -> Mux/2, Subsystem1/3(CCRB)
  Saturation2/1 -> Mux/3, Subsystem1/4(CCRC)
  Mux1/1 -> Scope2/1

== system huizhenglijujisuan_zuixin/current_loop/Subsystem ==
  Iabc : Inport
  θ : Inport  Port=2
  Clark : Subsystem
  Demux : Demux  Outputs=3
  "Park " : Subsystem
  iq : Outport  VectorParamsAs1DForOutWhenUnconnected=off
  id : Outport  Port=2  VectorParamsAs1DForOutWhenUnconnected=off
  tag scope: ialpha=global, ibeta=global
  wires:
  Demux/1 -> Clark/1(ia)
  Demux/3 -> Clark/3(ic)
  Demux/2 -> Clark/2(ib)
  Iabc/1 -> Demux/1
  θ/1 -> "Park "/3(Theta)
  Clark/2(ibeta) -> [ibeta], "Park "/2(ibeta)
  Clark/1(ialfa) -> [ialpha], "Park "/1(ialfa)
  "Park "/1(iq) -> iq/1
  "Park "/2(id) -> id/1

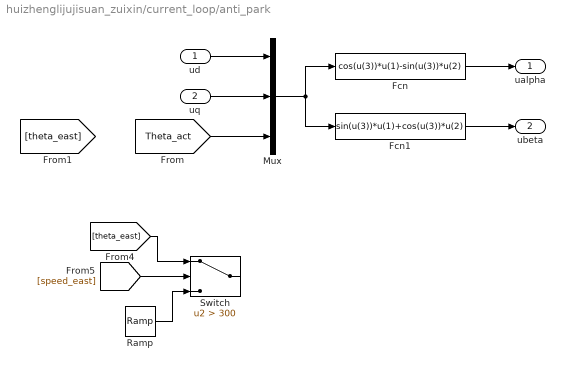
== system huizhenglijujisuan_zuixin/current_loop/anti_park ==
  ud : Inport
  uq : Inport  Port=2
  Fcn : Fcn  Expr=cos(u(3))*u(1)-sin(u(3))*u(2)
  Fcn1 : Fcn  Expr=sin(u(3))*u(1)+cos(u(3))*u(2)
  Mux : Mux  Inputs=3
  Ramp : simulink/Sources/Ramp  slope=50  start=0  InitialOutput=0
  Switch : Switch  Criteria=u2 > Threshold  Threshold=300  SaturateOnIntegerOverflow=off  InputSameDT=off
  ualpha : Outport
  ubeta : Outport  Port=2
  wires:
  Fcn/1 -> ualpha/1
  ud/1 -> Mux/1
  uq/1 -> Mux/2
  Fcn1/1 -> ubeta/1
  Mux/1 -> Fcn/1, Fcn1/1
  [theta_east] -> Switch/1
  Ramp/1 -> Switch/3
  [speed_east] -> Switch/2
  [Theta_act] -> Mux/3

== system huizhenglijujisuan_zuixin/alpha_lamda1/alpha/fl ==
  vx : Inport
  vy : Inport  Port=2
  wz : Inport  Port=3
  delta_fl : Inport  Port=4
  Add2 : Sum
  Add3 : Sum  Inputs=+-
  Add4 : Sum  Inputs=-+
  Divide : Product  Inputs=/*
  Gain3 : Gain  Gain=1.572
  Gain4 : Gain  Gain=0.5*1.7
  Trigonometric Function : Trigonometry  Operator=atan
  alpha_fl : Outport
  wires:
  Gain3/1 -> Add2/2
  Gain4/1 -> Add3/2
  Add2/1 -> Divide/2
  Add3/1 -> Divide/1
  Divide/1 -> Trigonometric Function/1
  Trigonometric Function/1 -> Add4/1
  vx/1 -> Add3/1
  delta_fl/1 -> Add4/2
  vy/1 -> Add2/1
  Add4/1 -> alpha_fl/1
  wz/1 -> Gain4/1, Gain3/1

== system huizhenglijujisuan_zuixin/alpha_lamda1/alpha/fr ==
  vx : Inport
  vy : Inport  Port=2
  wz : Inport  Port=3
  delta_fr : Inport  Port=4
  Add2 : Sum
  Add3 : Sum
  Add4 : Sum  Inputs=-+
  Divide : Product  Inputs=/*
  Gain3 : Gain  Gain=1.572
  Gain4 : Gain  Gain=0.5*1.7
  Trigonometric Function : Trigonometry  Operator=atan
  alpha_fr : Outport
  wires:
  Gain4/1 -> Add3/2
  wz/1 -> Gain3/1, Gain4/1
  Add4/1 -> alpha_fr/1
  vy/1 -> Add2/1
  delta_fr/1 -> Add4/2
  vx/1 -> Add3/1
  Trigonometric Function/1 -> Add4/1
  Divide/1 -> Trigonometric Function/1
  Add3/1 -> Divide/1
  Add2/1 -> Divide/2
  Gain3/1 -> Add2/2

== system huizhenglijujisuan_zuixin/alpha_lamda1/alpha/rl ==
  vx : Inport
  vy : Inport  Port=2
  wz : Inport  Port=3
  Add2 : Sum  Inputs=+-
  Add3 : Sum  Inputs=+-
  Divide : Product  Inputs=/*
  Gain3 : Gain  Gain=1.427
  Gain4 : Gain  Gain=0.5*1.7
  Trigonometric Function : Trigonometry  Operator=atan
  alpha_rl : Outport
  wires:
  Trigonometric Function/1 -> alpha_rl/1
  Gain4/1 -> Add3/2
  wz/1 -> Gain3/1, Gain4/1  "wz"
  vy/1 -> Add2/1  "vy"
  vx/1 -> Add3/1  "vx"
  Divide/1 -> Trigonometric Function/1
  Add3/1 -> Divide/1  "Vx_rl"
  Add2/1 -> Divide/2  "Vy_rl"
  Gain3/1 -> Add2/2

== system huizhenglijujisuan_zuixin/alpha_lamda1/alpha/rr ==
  vx : Inport
  vy : Inport  Port=2
  wz : Inport  Port=3
  Add2 : Sum  Inputs=+-
  Add3 : Sum
  Divide : Product  Inputs=/*
  Gain3 : Gain  Gain=1.427
  Gain4 : Gain  Gain=0.5*1.7
  Trigonometric Function : Trigonometry  Operator=atan
  alpha_rr : Outport
  wires:
  Trigonometric Function/1 -> alpha_rr/1
  Gain4/1 -> Add3/2
  Gain3/1 -> Add2/2
  Add2/1 -> Divide/2  "Vy_rr"
  Add3/1 -> Divide/1  "Vx_rr"
  Divide/1 -> Trigonometric Function/1
  vx/1 -> Add3/1  "vx"
  vy/1 -> Add2/1  "vy"
  wz/1 -> Gain4/1, Gain3/1  "wz"

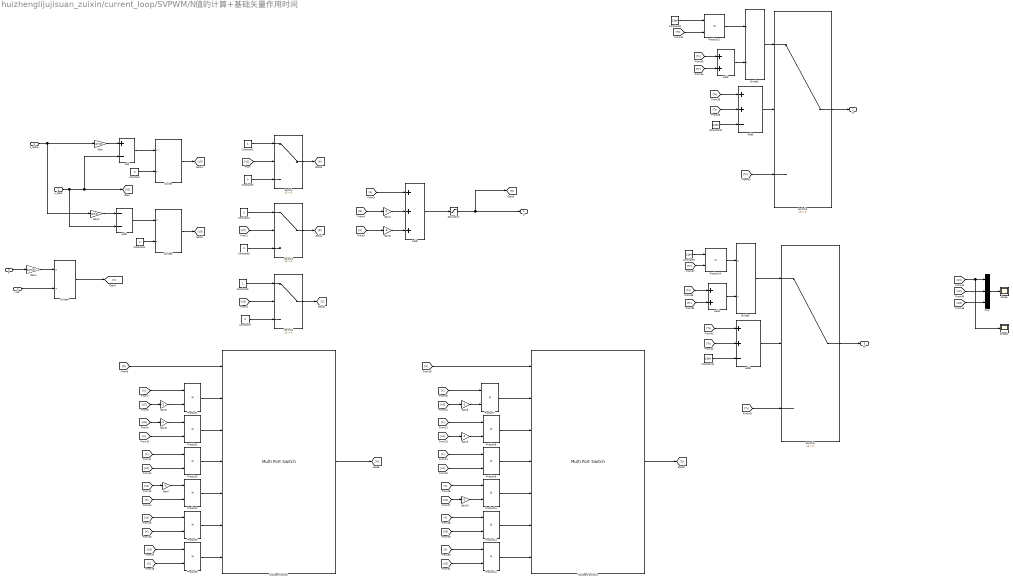
== system huizhenglijujisuan_zuixin/current_loop/SVPWM/N值的计算+基础矢量作用时间 ==
  u_alpha : Inport
  u_beta : Inport  Port=2
  T : Inport  Port=3
  Udc : Inport  Port=4
  Add : Sum  Inputs=+-
  Add1 : Sum  Inputs=--
  Add2 : Sum  Inputs=+++
  Add3 : Sum
  Add4 : Sum
  Add5 : Sum  Inputs=++-
  Add6 : Sum  Inputs=++-
  Constant : Constant  Value=2
  Constant1 : Constant  Value=2
  Constant{8..11} (4 alike) : Constant  Value=1/1e4
  Constant2 : Constant
  Constant3 : Constant  Value=0
  Constant4 : Constant
  Constant5 : Constant  Value=0
  Constant6 : Constant
  Constant7 : Constant  Value=0
  Divide{,1..4} (5 alike) : Product  Inputs=*/
  From3 : From
  Gain : Gain  Gain=sqrt(3)
  Gain1 : Gain  Gain=2
  Gain{5..10} (6 alike) : Gain  Gain=-1
  Gain2 : Gain  Gain=sqrt(3)
  Gain3 : Gain  Gain=4
  Gain4 : Gain  Gain=sqrt(3)
  Goto3 : Goto
  Multiport Switch : MultiPortSwitch  Inputs=6  SaturateOnIntegerOverflow=off  InputSameDT=off
  Multiport Switch1 : MultiPortSwitch  Inputs=6  SaturateOnIntegerOverflow=off  InputSameDT=off
  Mux : Mux  Inputs=3
  Product{1..14} (14 alike) : Product
  Saturation : Saturate  UpperLimit=6  LowerLimit=1
  Scope : Scope
  Scope1 : Scope
  Switch{,1..4} (5 alike) : Switch  Criteria=u2 > Threshold  SaturateOnIntegerOverflow=off  InputSameDT=off
  N : Outport
  Tx : Outport  Port=2
  Ty : Outport  Port=3
  wires:
  Switch4/1 -> Ty/1
  [Ty] -> Switch4/3
  Constant11/1 -> Add6/3
  [Ty] -> Add6/2
  [Tx] -> Add6/1
  Add6/1 -> Switch4/2
  Divide3/1 -> Switch4/1
  Switch3/1 -> Tx/1
  [Tx] -> Switch3/3
  Constant10/1 -> Add5/3
  [Ty] -> Add5/2
  [Tx] -> Add5/1
  Add5/1 -> Switch3/2
  Divide2/1 -> Switch3/1
  [Ty] -> Product14/2
  Constant9/1 -> Product14/1
  Product14/1 -> Divide3/1
  [Tx] -> Add4/1
  [Ty] -> Add4/2
  Add4/1 -> Divide3/2
  [Ty] -> Add3/2
  [Tx] -> Add3/1
  Add3/1 -> Divide2/2
  [Tx] -> Product13/2
  Constant8/1 -> Product13/1
  Product13/1 -> Divide2/1
  [U2] -> Product12/2
  [K] -> Product12/1
  Product12/1 -> Multiport Switch1/7
  [U3] -> Product11/2
  [K] -> Product11/1
  Product11/1 -> Multiport Switch1/6
  Gain10/1 -> Product10/2
  [U2] -> Gain10/1
  [K] -> Product10/1
  Product10/1 -> Multiport Switch1/5
  [U1] -> Product9/2
  [K] -> Product9/1
  Product9/1 -> Multiport Switch1/4
  Gain9/1 -> Product8/2
  [U1] -> Gain9/1
  [K] -> Product8/1
  Product8/1 -> Multiport Switch1/3
  Multiport Switch1/1 -> [Ty]
  Gain8/1 -> Product7/2
  [U3] -> Gain8/1
  [K] -> Product7/1
  Product7/1 -> Multiport Switch1/2
  [N] -> Multiport Switch1/1
  [K] -> Product6/2
  [U3] -> Product6/1
  Product6/1 -> Multiport Switch/7
  [K] -> Product5/2
  [U1] -> Product5/1
  Product5/1 -> Multiport Switch/6
  [K] -> Product4/2
  [U1] -> Gain7/1
  Gain7/1 -> Product4/1
  Product4/1 -> Multiport Switch/5
  [U2] -> Product3/2
  [K] -> Product3/1
  Product3/1 -> Multiport Switch/4
  [K] -> Product2/2
  Gain6/1 -> Product2/1
  [U3] -> Gain6/1
  Gain5/1 -> Product1/2
  Product2/1 -> Multiport Switch/3
  Multiport Switch/1 -> [Tx]
  [U2] -> Gain5/1
  [K] -> Product1/1
  Product1/1 -> Multiport Switch/2
  Udc/1 -> Divide4/2
  T/1 -> Gain4/1
  Gain4/1 -> Divide4/1
  Divide4/1 -> [K]
  [N] -> Multiport Switch/1
  Saturation/1 -> N/1, [N]
  Add2/1 -> Saturation/1
  [C] -> Gain3/1
  Gain3/1 -> Add2/3
  [B] -> Gain1/1
  Gain1/1 -> Add2/2
  From3/1 -> Add2/1
  Switch2/1 -> [C]
  Constant7/1 -> Switch2/3
  Constant6/1 -> Switch2/1
  [U3] -> Switch2/2
  Switch1/1 -> [B]
  Constant5/1 -> Switch1/3
  Constant4/1 -> Switch1/1
  [U2] -> Switch1/2
  Constant3/1 -> Switch/3
  Constant2/1 -> Switch/1
  Switch/1 -> Goto3/1
  [U1] -> Switch/2
  u_beta/1 -> [U1], Add/2, Add1/2
  Gain2/1 -> Add1/1
  Divide1/1 -> [U3]
  Constant1/1 -> Divide1/2
  Add1/1 -> Divide1/1
  Divide/1 -> [U2]
  Constant/1 -> Divide/2
  Add/1 -> Divide/1
  u_alpha/1 -> Gain/1, Gain2/1
  Gain/1 -> Add/1
  [U1] -> Scope1/1, Mux/1
  [U2] -> Mux/2
  [U3] -> Mux/3
  Mux/1 -> Scope/1

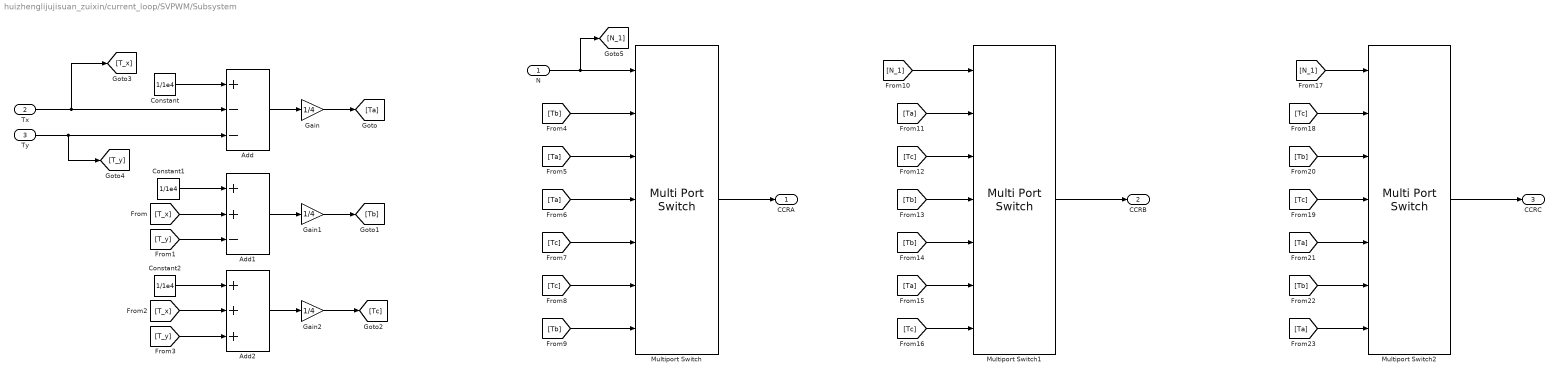
== system huizhenglijujisuan_zuixin/current_loop/SVPWM/Subsystem ==
  N : Inport
  Tx : Inport  Port=2
  Ty : Inport  Port=3
  Add : Sum  Inputs=+--
  Add1 : Sum  Inputs=++-
  Add2 : Sum  Inputs=+++
  Constant : Constant  Value=1/1e4
  Constant1 : Constant  Value=1/1e4
  Constant2 : Constant  Value=1/1e4
  Gain : Gain  Gain=1/4
  Gain1 : Gain  Gain=1/4
  Gain2 : Gain  Gain=1/4
  Multiport Switch : MultiPortSwitch  Inputs=6  SaturateOnIntegerOverflow=off  InputSameDT=off
  Multiport Switch1 : MultiPortSwitch  Inputs=6  SaturateOnIntegerOverflow=off  InputSameDT=off
  Multiport Switch2 : MultiPortSwitch  Inputs=6  SaturateOnIntegerOverflow=off  InputSameDT=off
  CCRA : Outport
  CCRB : Outport  Port=2
  CCRC : Outport  Port=3
  wires:
  [Ta] -> Multiport Switch2/7
  [Tb] -> Multiport Switch2/6
  [Ta] -> Multiport Switch2/5
  [Tc] -> Multiport Switch2/4
  [Tb] -> Multiport Switch2/3
  [Tc] -> Multiport Switch2/2
  Multiport Switch2/1 -> CCRC/1
  [N_1] -> Multiport Switch2/1
  [Tc] -> Multiport Switch1/7
  [Ta] -> Multiport Switch1/6
  [Tb] -> Multiport Switch1/5
  [Tb] -> Multiport Switch1/4
  [Tc] -> Multiport Switch1/3
  [Ta] -> Multiport Switch1/2
  Multiport Switch1/1 -> CCRB/1
  [N_1] -> Multiport Switch1/1
  [Tb] -> Multiport Switch/7
  [Tc] -> Multiport Switch/6
  [Tc] -> Multiport Switch/5
  [Ta] -> Multiport Switch/4
  [Ta] -> Multiport Switch/3
  [Tb] -> Multiport Switch/2
  Multiport Switch/1 -> CCRA/1
  N/1 -> Multiport Switch/1, [N_1]
  [T_y] -> Add2/3
  [T_x] -> Add2/2
  Constant2/1 -> Add2/1
  Gain2/1 -> [Tc]
  Add2/1 -> Gain2/1
  Gain1/1 -> [Tb]
  Add1/1 -> Gain1/1
  [T_y] -> Add1/3
  [T_x] -> Add1/2
  Constant1/1 -> Add1/1
  Gain/1 -> [Ta]
  Add/1 -> Gain/1
  Ty/1 -> Add/3, [T_y]
  Tx/1 -> Add/2, [T_x]
  Constant/1 -> Add/1

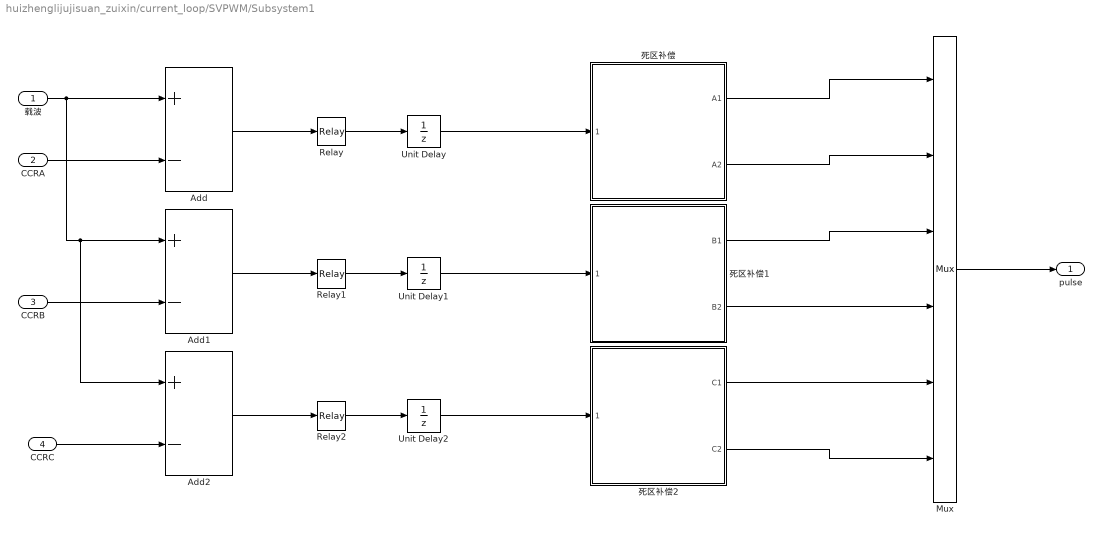
== system huizhenglijujisuan_zuixin/current_loop/SVPWM/Subsystem1 ==
  载波 : Inport
  CCRA : Inport  Port=2
  CCRB : Inport  Port=3
  CCRC : Inport  Port=4
  Add : Sum  Inputs=+-
  Add1 : Sum  Inputs=+-
  Add2 : Sum  Inputs=+-
  Mux : Mux  Inputs=6
  Relay : Relay
  Relay1 : Relay
  Relay2 : Relay
  Unit Delay : UnitDelay  SampleTime=-1  HasFrameUpgradeWarning=on
  Unit Delay1 : UnitDelay  SampleTime=-1  HasFrameUpgradeWarning=on
  Unit Delay2 : UnitDelay  SampleTime=-1  HasFrameUpgradeWarning=on
  死区补偿 : Subsystem
  死区补偿1 : Subsystem
  死区补偿2 : Subsystem
  pulse : Outport
  wires:
  Mux/1 -> pulse/1
  死区补偿2/2(C2) -> Mux/6
  死区补偿2/1(C1) -> Mux/5
  死区补偿1/2(B2) -> Mux/4
  死区补偿1/1(B1) -> Mux/3
  死区补偿/2(A2) -> Mux/2
  死区补偿/1(A1) -> Mux/1
  Unit Delay2/1 -> 死区补偿2/1(1)
  Unit Delay1/1 -> 死区补偿1/1(1)
  Unit Delay/1 -> 死区补偿/1(1)
  Relay2/1 -> Unit Delay2/1
  Relay1/1 -> Unit Delay1/1
  Relay/1 -> Unit Delay/1
  Add2/1 -> Relay2/1
  Add1/1 -> Relay1/1
  Add/1 -> Relay/1
  CCRC/1 -> Add2/2
  CCRB/1 -> Add1/2
  CCRA/1 -> Add/2
  载波/1 -> Add/1, Add1/1, Add2/1

== system huizhenglijujisuan_zuixin/current_loop/Subsystem/Clark ==
  ia : Inport
  ib : Inport  Port=2
  ic : Inport  Port=3
  Fcn : Fcn  Expr=2/3*(u[1]-0.5*u[2]-0.5*u[3])
  Fcn1 : Fcn  Expr=2/3*(sqrt(3/4)*u(2)-sqrt(3/4)*u(3))
  Mux : Mux  Inputs=3
  ialfa : Outport  VectorParamsAs1DForOutWhenUnconnected=off
  ibeta : Outport  Port=2  VectorParamsAs1DForOutWhenUnconnected=off
  wires:
  ic/1 -> Mux/3
  Fcn1/1 -> ibeta/1
  Fcn/1 -> ialfa/1
  Mux/1 -> Fcn1/1, Fcn/1
  ib/1 -> Mux/2
  ia/1 -> Mux/1

== system huizhenglijujisuan_zuixin/current_loop/Subsystem/Park  ==
  ialfa : Inport
  ibeta : Inport  Port=2
  Theta : Inport  Port=3
  Fcn : Fcn  Expr=u(2)*cos(u(3))-u(1)*sin(u(3))
  Fcn1 : Fcn  Expr=u(2)*sin(u(3))+u(1)*cos(u(3))
  Mux : Mux  Inputs=3
  iq : Outport  VectorParamsAs1DForOutWhenUnconnected=off
  id : Outport  Port=2  VectorParamsAs1DForOutWhenUnconnected=off
  wires:
  Theta/1 -> Mux/3
  Fcn1/1 -> id/1
  Fcn/1 -> iq/1
  Mux/1 -> Fcn/1, Fcn1/1
  ibeta/1 -> Mux/2
  ialfa/1 -> Mux/1

== system huizhenglijujisuan_zuixin/current_loop/SVPWM/Subsystem1/死区补偿 ==
  1 : Inport
  Abs : Abs  SaturateOnIntegerOverflow=off
  Add : Sum  Inputs=+-
  Data Type Conversion : DataTypeConversion  OutDataTypeStr=double  SaturateOnIntegerOverflow=off  RndMeth=Floor
  Logical Operator : Logic  Operator=NOT  AllPortsSameDT=off  OutDataTypeStr=boolean
  Product : Product
  Product1 : Product
  Transport Delay : TransportDelay  DelayTime=0
  A1 : Outport
  A2 : Outport  Port=2
  wires:
  Abs/1 -> Product1/2, Product/1
  Product1/1 -> A1/1
  Add/1 -> Abs/1
  Product/1 -> A2/1
  Transport Delay/1 -> Product/2, Add/2
  Data Type Conversion/1 -> Transport Delay/1
  Logical Operator/1 -> Data Type Conversion/1
  1/1 -> Logical Operator/1, Add/1, Product1/1

== system huizhenglijujisuan_zuixin/current_loop/SVPWM/Subsystem1/死区补偿1 ==
  1 : Inport
  Abs : Abs  SaturateOnIntegerOverflow=off
  Add : Sum  Inputs=+-
  Data Type Conversion : DataTypeConversion  OutDataTypeStr=double  SaturateOnIntegerOverflow=off  RndMeth=Floor
  Logical Operator : Logic  Operator=NOT  AllPortsSameDT=off  OutDataTypeStr=boolean
  Product : Product
  Product1 : Product
  Transport Delay : TransportDelay  DelayTime=0
  B1 : Outport
  B2 : Outport  Port=2
  wires:
  1/1 -> Product1/1, Add/1, Logical Operator/1
  Logical Operator/1 -> Data Type Conversion/1
  Data Type Conversion/1 -> Transport Delay/1
  Transport Delay/1 -> Add/2, Product/2
  Product/1 -> B2/1
  Add/1 -> Abs/1
  Product1/1 -> B1/1
  Abs/1 -> Product/1, Product1/2

== system huizhenglijujisuan_zuixin/current_loop/SVPWM/Subsystem1/死区补偿2 ==
  1 : Inport
  Abs : Abs  SaturateOnIntegerOverflow=off
  Add : Sum  Inputs=+-
  Data Type Conversion : DataTypeConversion  OutDataTypeStr=double  SaturateOnIntegerOverflow=off  RndMeth=Floor
  Logical Operator : Logic  Operator=NOT  AllPortsSameDT=off  OutDataTypeStr=boolean
  Product : Product
  Product1 : Product
  Transport Delay : TransportDelay  DelayTime=0
  C1 : Outport
  C2 : Outport  Port=2
  wires:
  Abs/1 -> Product1/2, Product/1
  Product1/1 -> C1/1
  Add/1 -> Abs/1
  Product/1 -> C2/1
  Transport Delay/1 -> Product/2, Add/2
  Data Type Conversion/1 -> Transport Delay/1
  Logical Operator/1 -> Data Type Conversion/1
  1/1 -> Logical Operator/1, Add/1, Product1/1

== matlab function huizhenglijujisuan_zuixin/PAC1/fr ==
  data: Fz input; alpha input; Fy0 output; Mz output; t output; Mzr output; M1 output; Mznew output
function [Fy0,Mz,t,Mzr,M1,Mznew] = tire(Fz,alpha)
t=0;
Mzr=0;
if Fz>0
%Fz 轮胎垂向载荷 N
%camber 外倾角 rad？？？
%lamda 纵向滑移率
%alpha 车辆侧偏角 rad
alpha=tan(alpha);
camber=0;
Fz0=8000; %名义垂向载荷N
dfz=(Fz-Fz0)/Fz0;
% %% Pure_Fx
% %轮胎参数——纵向力
% pcx1=1.65;
% pdx1=1.3; pdx2=-0.15; pdx3=0;
% pex1=0; pex2=0;pex3=0; pex4=0;
% pkx1=20; pkx2=0; pkx3=0;
% pvx1=0; pvx2=0;
% phx1=0; phx2=0;
% %pure_Fx 魔术公式
% Cx=pcx1;
% Shx=phx1+phx2*dfz;
% lamda_x=lamda+Shx;
% Dx=(pdx1+pdx2*dfz)*(1-pdx3*camber*camber)*Fz;
% Ex=(pex1+pex2*dfz+pex3*dfz*dfz)*(1-pex4*sign(lamda_x));
% Kx=Fz*(pkx1+pkx2*dfz)*exp(pkx3*dfz);
% Bx=Kx/(Cx*Dx);
% Svx=Fz*(pvx1+pvx2*dfz);
% Fx0=Dx*sin(Cx*atan(Bx*lamda_x-Ex*(Bx*lamda_x-atan(Bx*lamda_x))))+Svx;
% %% 联合工况纵向力Fx
% %轮胎参数——纵向力
% rbx1=20;rbx2=15;
% rcx1=1;
% rex1=0;rex2=0;
% rhx1=0;
% %纵向力加权函数
% Bxa=rbx1*cos(atan(rbx2*lamda));
% Cxa=rcx1;
% Exa=rex1+rex2*dfz;
% Shxa=rhx1;
% alpha_s=alpha+Shxa;
% Gxa=cos(Cxa*atan(Bxa*alpha_s-Exa*(Bxa*alpha_s-atan(Bxa*alpha_s))))/cos(Cxa*atan(Bxa*Shxa-Exa*(Bxa*Shxa-atan(Bxa*Shxa))));
% Fx=Fx0*Gxa;



%% Pure_Fy
%轮胎参数——侧向力
pcy1=1.529245171;
pdy1=1.038581713; pdy2=-0.179464279; pdy3=-0.683745879;
pey1=-0.39012519; pey2=-0.611160145;pey3=-0.040677215; pey4=-14.95422065;
pky1=-26.056726760; pky2=2.106504624; pky3=0.499984439;
pvy1=0; pvy2=0;pvy3=0;pvy4=0;
phy1=0; phy2=0;phy3=0;
%pure_Fy 魔术公式
Cy=pcy1;
Shy=phy1+phy2*dfz+phy3*camber;
alpha_y=alpha+Shy;
uy=(pdy1+pdy2*dfz)*(1-pdy3*camber*camber);
Dy=uy*Fz;
Ey=(pey1+pey2*dfz)*(1-(pey3+pey4*camber)*sign(alpha_y));
Ky=pky1*Fz0*sin(2*atan(Fz/(pky2*Fz0)))*(1-pky3*abs(camber));
By=Ky/(Cy*Dy);
Svy=Fz*(pvy1+pvy2*dfz+(pvy3+pvy4*dfz)*camber);
Fy0=Dy*sin(Cy*atan(By*alpha_y-Ey*(By*alpha_y-atan(By*alpha_y))))+Svy;
% %% 联合工况侧向力Fy
% %轮胎参数——侧向力
% rby1=10;rby2=10;rby3=-0.027856;
% rcy1=1;
% rey1=0;rey2=0;
% rhy1=0;rhy2=0;
% rvy1=0;rvy2=0;rvy3=0;rvy4=20;rvy5=2;rvy6=10;
% %侧向力加权函数
% Bya=rby1*cos(atan(rby2*(alpha-rby3)));
% Cya=rcy1;
% Eya=rey1+rey2*dfz;
% Shya=rhy1+rhy2*dfz;
% lamda_s=lamda+Shya;
% Gya=cos(Cya*atan(Bya*lamda_s-Eya*(Bya*lamda_s-atan(Bya*lamda_s))))/cos(Cya*atan(Bya*Shya-Eya*(Bya*Shya-atan(Bya*Shya))));
% %轮胎参数——侧向力
% Svyr=uy*Fz*(rvy1+rvy2*dfz+rvy3*camber)*cos(atan(rvy4*alpha))*sin(rvy5*atan(rvy6*lamda));
% Fy=Fy0*Gya+Svyr;

%% Pure_Mz
%轮胎参数——回正力矩
R0=0.357; %轮胎空载半径/m
qbz1=8.37;qbz2=-2.92;qbz3=0.48;qbz4=-0.45;qbz5=-0.44;
qcz1=1.19;
qdz1=0.11;qdz2=-0.003;qdz3=-0.56;qdz4=8.4;
qez1=-2.9;qez2=-0.55;qez3=0;qez4=-0.13;qez5=-3.68;
%pure_Mz0 魔术公式
Ct=qcz1;
alpha_t=alpha;
Bt=(qbz1+qbz2*dfz+qbz3*dfz^2)*(1+qbz4*camber+qbz5*abs(camber));
Dt=Fz*(qdz1+qdz2*dfz)*(1+qdz3*camber+qdz4*camber^2)*R0/Fz0;
Et=(qez1+qez2*dfz+qez3*dfz^2)*(1+(qez4+qez5*camber)*((2/pi)*atan(Bt*Ct*alpha_t)));
t=Dt*cos(Ct*atan(Bt*alpha_t-Et*(Bt*alpha_t-atan(Bt*alpha_t))))*cos(alpha); %轮胎拖距
% 轮胎参数——回正力矩
qbz9=3.44;qbz10=0;
qdz6=0.003;qdz7=0.005;qdz8=-0.12;qdz9=0.12;
Br=(qbz9+qbz10*By*Cy);
Cr=1;
Dr=Fz*(qdz6+qdz7*dfz+(qdz8+qdz9*dfz)*camber)*R0;
alpha_r=alpha;
Mzr=Dr*cos(Cr*atan(Br*alpha_r))*cos(alpha); %残余力矩
M1=-R0*tan(5/180*pi)*Fy0;
Mz=-t*Fy0;
Mznew=Mz+M1;
else
    Fx0=0;
    Fy0=0;
    Fx=0;
    Fy=0;
    Mz=0;
    M1=0;
    Mznew=0;
end

== matlab function huizhenglijujisuan_zuixin/PAC1/rl ==
  data: Fz input; alpha input; Fy0 output; Mz output
function [Fy0,Mz] = tire(Fz,alpha)
if Fz>0
%Fz 轮胎垂向载荷 N
%camber 外倾角 rad？？？
%lamda 纵向滑移率
%alpha 车辆侧偏角 rad
alpha=tan(alpha);
camber=0;
Fz0=8000; %名义垂向载荷N
dfz=(Fz-Fz0)/Fz0;
% %% Pure_Fx
% %轮胎参数——纵向力
% pcx1=1.65;
% pdx1=1.3; pdx2=-0.15; pdx3=0;
% pex1=0; pex2=0;pex3=0; pex4=0;
% pkx1=20; pkx2=0; pkx3=0;
% pvx1=0; pvx2=0;
% phx1=0; phx2=0;
% %pure_Fx 魔术公式
% Cx=pcx1;
% Shx=phx1+phx2*dfz;
% lamda_x=lamda+Shx;
% Dx=(pdx1+pdx2*dfz)*(1-pdx3*camber*camber)*Fz;
% Ex=(pex1+pex2*dfz+pex3*dfz*dfz)*(1-pex4*sign(lamda_x));
% Kx=Fz*(pkx1+pkx2*dfz)*exp(pkx3*dfz);
% Bx=Kx/(Cx*Dx);
% Svx=Fz*(pvx1+pvx2*dfz);
% Fx0=Dx*sin(Cx*atan(Bx*lamda_x-Ex*(Bx*lamda_x-atan(Bx*lamda_x))))+Svx;
% %% 联合工况纵向力Fx
% %轮胎参数——纵向力
% rbx1=20;rbx2=15;
% rcx1=1;
% rex1=0;rex2=0;
% rhx1=0;
% %纵向力加权函数
% Bxa=rbx1*cos(atan(rbx2*lamda));
% Cxa=rcx1;
% Exa=rex1+rex2*dfz;
% Shxa=rhx1;
% alpha_s=alpha+Shxa;
% Gxa=cos(Cxa*atan(Bxa*alpha_s-Exa*(Bxa*alpha_s-atan(Bxa*alpha_s))))/cos(Cxa*atan(Bxa*Shxa-Exa*(Bxa*Shxa-atan(Bxa*Shxa))));
% Fx=Fx0*Gxa;



%% Pure_Fy
%轮胎参数——侧向力
pcy1=1.529245171;
pdy1=1.038581713; pdy2=-0.179464279; pdy3=-0.683745879;
pey1=-0.39012519; pey2=-0.611160145;pey3=-0.040677215; pey4=-14.95422065;
pky1=-26.056726760; pky2=2.106504624; pky3=0.499984439;
pvy1=0; pvy2=0;pvy3=0;pvy4=0;
phy1=0; phy2=0;phy3=0;
%pure_Fy 魔术公式
Cy=pcy1;
Shy=phy1+phy2*dfz+phy3*camber;
alpha_y=alpha+Shy;
uy=(pdy1+pdy2*dfz)*(1-pdy3*camber*camber);
Dy=uy*Fz;
Ey=(pey1+pey2*dfz)*(1-(pey3+pey4*camber)*sign(alpha_y));
Ky=pky1*Fz0*sin(2*atan(Fz/(pky2*Fz0)))*(1-pky3*abs(camber));
By=Ky/(Cy*Dy);
Svy=Fz*(pvy1+pvy2*dfz+(pvy3+pvy4*dfz)*camber);
Fy0=Dy*sin(Cy*atan(By*alpha_y-Ey*(By*alpha_y-atan(By*alpha_y))))+Svy;
% %% 联合工况侧向力Fy
% %轮胎参数——侧向力
% rby1=10;rby2=10;rby3=-0.027856;
% rcy1=1;
% rey1=0;rey2=0;
% rhy1=0;rhy2=0;
% rvy1=0;rvy2=0;rvy3=0;rvy4=20;rvy5=2;rvy6=10;
% %侧向力加权函数
% Bya=rby1*cos(atan(rby2*(alpha-rby3)));
% Cya=rcy1;
% Eya=rey1+rey2*dfz;
% Shya=rhy1+rhy2*dfz;
% lamda_s=lamda+Shya;
% Gya=cos(Cya*atan(Bya*lamda_s-Eya*(Bya*lamda_s-atan(Bya*lamda_s))))/cos(Cya*atan(Bya*Shya-Eya*(Bya*Shya-atan(Bya*Shya))));
% %轮胎参数——侧向力
% Svyr=uy*Fz*(rvy1+rvy2*dfz+rvy3*camber)*cos(atan(rvy4*alpha))*sin(rvy5*atan(rvy6*lamda));
% Fy=Fy0*Gya+Svyr;

%% Pure_Mz
%轮胎参数——回正力矩
R0=0.357; %轮胎空载半径/m
qbz1=8.37;qbz2=-2.92;qbz3=0.48;qbz4=-0.45;qbz5=-0.44;
qcz1=1.19;
qdz1=0.11;qdz2=-0.003;qdz3=-0.56;qdz4=8.4;
qez1=-2.9;qez2=-0.55;qez3=0;qez4=-0.13;qez5=-3.68;
%pure_Mz0 魔术公式
Ct=qcz1;
alpha_t=alpha;
Bt=(qbz1+qbz2*dfz+qbz3*dfz^2)*(1+qbz4*camber+qbz5*abs(camber));
Dt=Fz*(qdz1+qdz2*dfz)*(1+qdz3*camber+qdz4*camber^2)*R0/Fz0;
Et=(qez1+qez2*dfz+qez3*dfz^2)*(1+(qez4+qez5*camber)*((2/pi)*atan(Bt*Ct*alpha_t)));
t=Dt*cos(Ct*atan(Bt*alpha_t-Et*(Bt*alpha_t-atan(Bt*alpha_t))))*cos(alpha); %轮胎拖距
% 轮胎参数——回正力矩
qbz9=3.44;qbz10=0;
qdz6=0.003;qdz7=0.005;qdz8=-0.12;qdz9=0.12;
Br=(qbz9+qbz10*By*Cy);
Cr=1;
Dr=Fz*(qdz6+qdz7*dfz+(qdz8+qdz9*dfz)*camber)*R0;
alpha_r=alpha;
Mzr=Dr*cos(Cr*atan(Br*alpha_r))*cos(alpha); %残余力矩
Mz=-t*Fy0+Mzr;
else
    Fx0=0;
    Fy0=0;
    Fx=0;
    Fy=0;
    Mz=0;
end
